simulink library "syntrac_lib"  (R2023b)
settings: Solver=VariableStepAuto  StartTime=0.0  StopTime=10.0  RelTol=1e-3
undefined symbols (not defined in the file or in its folder): aircraft, ic
libraries: unit_conversions_lib x9, actuators_lib x5, vlm_wing_lib x3, flight_parameters_lib x1, axes_transformation_lib x1, rigidBody_lib x1
settings Model: Creator=yannic  LastModifiedBy=Ole Bunde

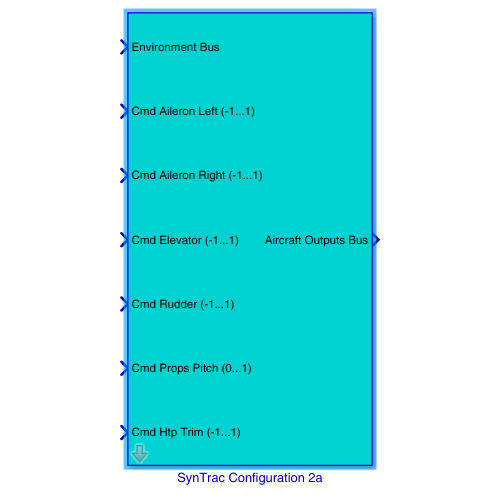
[thumbnail: Simulink's stored preview of the top-level diagram]
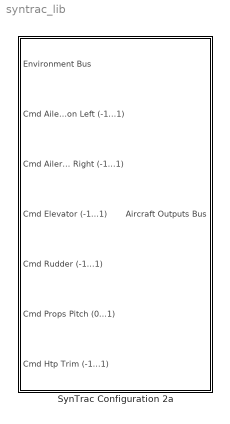
== system syntrac_lib ==
  SynTrac Configuration 2a : Subsystem  mask{aircraft=aircraft, ic=ic}
      mask prompts: aircraft "Aircraft parameters struct, see aircraftSe2aCreate"; ic "Initial conditions struct"
      mask init:
      | aircraft_state = aircraftSyntracGetState(aircraft);
      | struct2bus(aircraft_state);
      mask DialogControl DescGroupVar Prompt: Rigid aircraft with steady aerodynamics
      mask DialogControl DescTextVar Prompt: Rigid-body equations of motion, steady aerodynamics based on nonlinear lifting-line method.

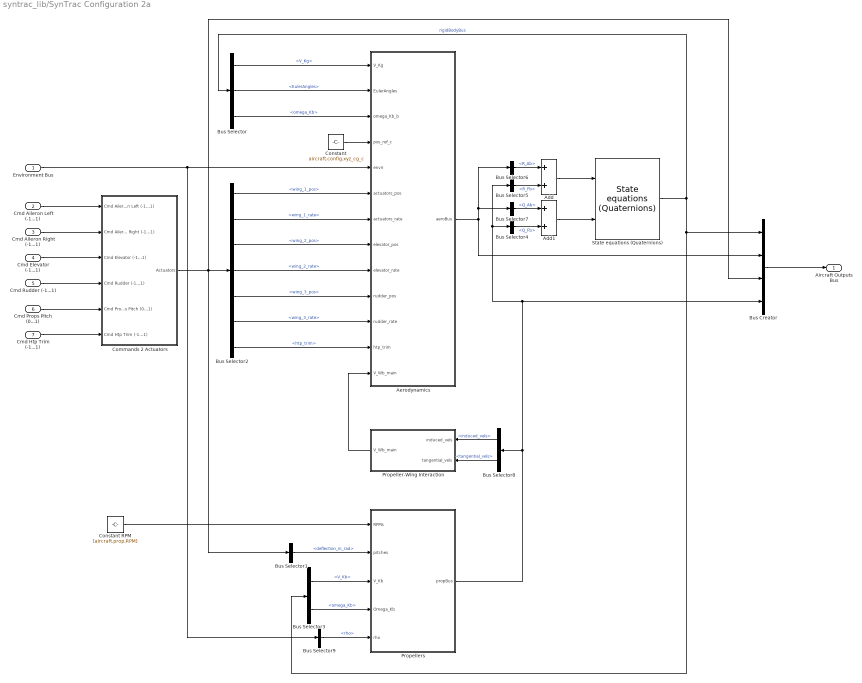
== system syntrac_lib/SynTrac Configuration 2a ==
  Environment Bus : Inport
  Cmd Aileron Left (-1...1) : Inport  Port=2
  Cmd Aileron Right (-1...1) : Inport  Port=3
  Cmd Elevator (-1...1) : Inport  Port=4
  Cmd Rudder (-1...1) : Inport  Port=5
  Cmd Props Pitch (0...1) : Inport  Port=6
  Cmd Htp Trim (-1...1) : Inport  Port=7
  Add : Sum
  Add1 : Sum
  Aerodynamics : Subsystem
  Bus Creator : BusCreator  Inputs=4
  Bus Selector : BusSelector  OutputSignals=V_Kg,EulerAngles,omega_Kb
  Bus Selector1 : BusSelector  OutputSignals=props_pitch.deflection_in_rad
  Bus Selector2 : BusSelector  OutputSignals=wing_1_pos,wing_1_rate,wing_2_pos,wing_2_rate,wing_3_pos,wing_3_rate,htp_trim
  Bus Selector3 : BusSelector  OutputSignals=V_Kb,omega_Kb
  Bus Selector4 : BusSelector  OutputSignals=Q_Fb
  Bus Selector5 : BusSelector  OutputSignals=R_Fb
  Bus Selector6 : BusSelector  OutputSignals=R_Ab
  Bus Selector7 : BusSelector  OutputSignals=Q_Ab
  Bus Selector8 : BusSelector  OutputSignals=induced_vels,tangential_vels
  Bus Selector9 : BusSelector  OutputSignals=atmosphere.rho
  Commands 2 Actuators : Subsystem  mask{aileron=aircraft.actuators.aileron, elevator=aircraft.actuators.elevator, rudder=aircraft.actuators.rudder, prop=aircraft.actuators.prop_pitch, htp_trim=aircraft.actuators.htp_trim, ic=ic.act}
      mask prompts: aileron "Aileron parameters"; elevator "Elevator parameters"; rudder "Rudder parameters"; prop "Engines parameters"; htp_trim "Trimmable horizontal tailplane (htp) parameters"; ic "Initial conditions struct"
      mask DialogControl DescGroupVar Prompt: SE2A Actuator Dynamics
      mask DialogControl DescTextVar Prompt: Input commands are defined as bus.
  Constant : Constant  Value=aircraft.config.xyz_cg_c
  Constant RPM : Constant  Value=[aircraft.prop.RPM]
  Propeller-Wing Interaction : Subsystem  mask{prop=aircraft.prop, wing=aircraft.wing_main}
      mask prompts: prop "Propeller struct"; wing "Wing struct"
  Propellers : Subsystem  mask{prop=aircraft.prop, prop_map=aircraft.prop_table, pos_cg_c=aircraft.config.xyz_cg_c}
      mask prompts: prop "Array of propeller structs"; prop_map "Propeller map struct"; pos_cg_c "Center of gravity positions in c frame, m"
      mask init:
      | num_props = length(prop);
      |     M_bp = zeros(3,3,num_props);
      |     r_p_b = zeros(3,num_props);
      |     for i = 1:num_props
      |         M_bp(:,:,i) = [ ...
      |             cos(prop(i).angle),0,sin(prop(i).angle); ...
      |             0,1,0; ...
      |             -sin(prop(i).angle),0,cos(prop(i).angle) ...
      |             ];
      |         r_p_b(:,i) = prop(i).pos_c - pos_cg_c;
      |     end
      |     prop_ang = [prop.angle];
  State equations (Quaternions) : rigidBody_lib/State equations (Quaternions)  m=aircraft.body.m  I=aircraft.body.I  is_g_checked=off  g=9.81  omega_Kb_0=ic.omega_Kb  q_bg_0=ic.q_bg  V_Kb_0=ic.V_Kb  s_g_0=ic.s_Kg
      settings: SourceProductName=LADAC
  Aircraft Outputs Bus : Outport  VectorParamsAs1DForOutWhenUnconnected=off
  wires:
  Add/1 -> State equations (Quaternions)/1
  Environment Bus/1 -> Aerodynamics/5(envir), Bus Selector9/1
  State equations (Quaternions)/1 -> Bus Creator/1, Bus Selector3/1, Bus Selector/1  "rigidBodyBus"
  Bus Selector/1 -> Aerodynamics/1(V_Kg)  "<V_Kg>"
  Bus Selector/2 -> Aerodynamics/2(EulerAngles)  "<EulerAngles>"
  Bus Selector/3 -> Aerodynamics/3(omega_Kb_b)  "<omega_Kb>"
  Bus Creator/1 -> Aircraft Outputs Bus/1
  Bus Selector2/6 -> Aerodynamics/11(rudder_rate)  "<wing_3_rate>"
  Bus Selector2/7 -> Aerodynamics/12(htp_trim)  "<htp_trim>"
  Bus Selector2/3 -> Aerodynamics/8(elevator_pos)  "<wing_2_pos>"
  Bus Selector2/2 -> Aerodynamics/7(actuators_rate)  "<wing_1_rate>"
  Cmd Aileron Left (-1...1)/1 -> Commands 2 Actuators/1(Cmd Aileron Left (-1...1))
  Bus Selector2/1 -> Aerodynamics/6(actuators_pos)  "<wing_1_pos>"
  Bus Selector2/5 -> Aerodynamics/10(rudder_pos)  "<wing_3_pos>"
  Bus Selector2/4 -> Aerodynamics/9(elevator_rate)  "<wing_2_rate>"
  Constant/1 -> Aerodynamics/4(pos_ref_c)
  Commands 2 Actuators/1(Actuators) -> Bus Selector1/1, Bus Creator/3, Bus Selector2/1
  Cmd Aileron Right (-1...1)/1 -> Commands 2 Actuators/2(Cmd Aileron Right (-1...1))
  Cmd Elevator (-1...1)/1 -> Commands 2 Actuators/3(Cmd Elevator (-1...1))
  Cmd Rudder (-1...1)/1 -> Commands 2 Actuators/4(Cmd Rudder (-1...1))
  Cmd Props Pitch (0...1)/1 -> Commands 2 Actuators/5(Cmd Props Pitch (0...1))
  Cmd Htp Trim (-1...1)/1 -> Commands 2 Actuators/6(Cmd Htp Trim (-1...1))
  Constant RPM/1 -> Propellers/1(RPMs)
  Bus Selector1/1 -> Propellers/2(pitches)  "<deflection_in_rad>"
  Bus Selector3/1 -> Propellers/3(V_Kb)  "<V_Kb>"
  Bus Selector3/2 -> Propellers/4(Omega_Kb)  "<omega_Kb>"
  Add1/1 -> State equations (Quaternions)/2
  Propellers/1(propBus) -> Bus Selector5/1, Bus Selector4/1, Bus Creator/4, Bus Selector8/1
  Bus Selector5/1 -> Add/2  "<R_Fb>"
  Bus Selector4/1 -> Add1/2  "<Q_Fb>"
  Bus Selector6/1 -> Add/1  "<R_Ab>"
  Bus Selector7/1 -> Add1/1  "<Q_Ab>"
  Aerodynamics/1(aeroBus) -> Bus Creator/2, Bus Selector7/1, Bus Selector6/1
  Bus Selector8/1 -> Propeller-Wing Interaction/1(induced_vels)  "<induced_vels>"
  Bus Selector9/1 -> Propellers/5(rho)  "<rho>"
  Bus Selector8/2 -> Propeller-Wing Interaction/2(tangential_vels)  "<tangential_vels>"
  Propeller-Wing Interaction/1(V_Wb_main) -> Aerodynamics/13(V_Wb_main)

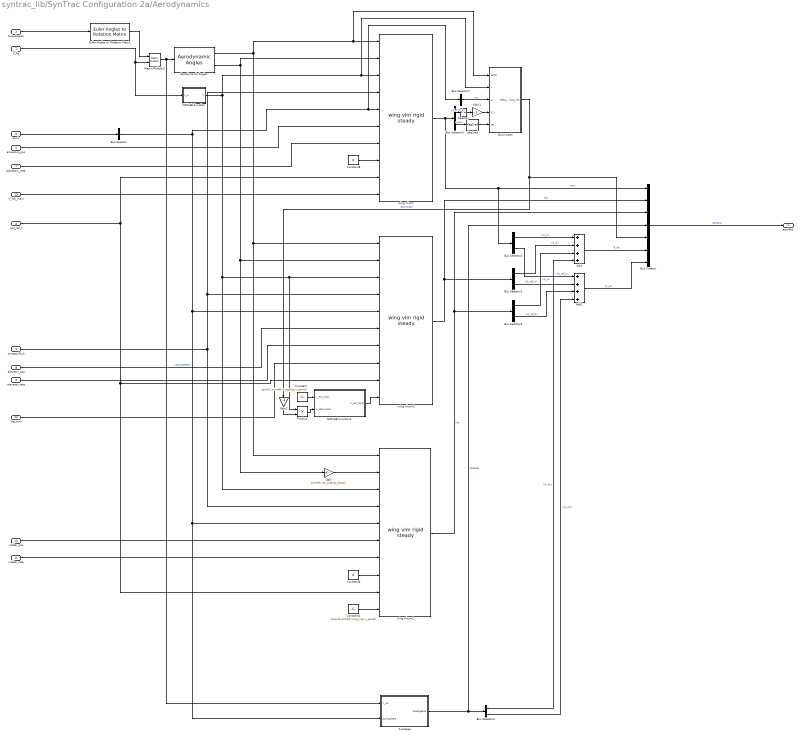
== system syntrac_lib/SynTrac Configuration 2a/Aerodynamics ==
  V_Kg : Inport
  EulerAngles : Inport  Port=2
  omega_Kb_b : Inport  Port=3
  pos_ref_c : Inport  Port=4
  envir : Inport  Port=5
  actuators_pos : Inport  Port=6
  actuators_rate : Inport  Port=7
  elevator_pos : Inport  Port=8
  elevator_rate : Inport  Port=9
  rudder_pos : Inport  Port=10
  rudder_rate : Inport  Port=11
  htp_trim : Inport  Port=12
  V_Wb_main : Inport  Port=13
  Add : Sum  Inputs=++++
  Add1 : Sum  Inputs=++++
  Aerodynamic Angles : flight_parameters_lib/Aerodynamic Angles  SystemSampleTime=-1  VariantActivationTime=update diagram  AllowFlexibleInterface=on  Latency=0  AutoFrameSizeCalculation=off
      settings: SourceProductName=LADAC
  Bus Creator : BusCreator  Inputs=7
  Bus Selector : BusSelector  OutputSignals=atmosphere
  Bus Selector1 : BusSelector  OutputSignals=aero.force_glob.R_b,aero.force_glob.Q_ref_b
  Bus Selector2 : BusSelector  OutputSignals=aero.force_glob.R_b,aero.force_glob.Q_ref_b
  Bus Selector3 : BusSelector  OutputSignals=aero.force_glob.R_b,aero.force_glob.Q_ref_b
  Bus Selector4 : BusSelector  OutputSignals=R_Ab,Q_Ab
  Bus Selector5 : BusSelector  OutputSignals=aero.coeff_glob.C_XYZ_b,actuators.pos
  Bus Selector7 : BusSelector  OutputSignals=a
  Constant : Constant  Value=zeros(3,aircraft.wing_htp.n_panel)
  Constant2 : Constant  Value=zeros(3,aircraft.wing_vtp.n_panel)
  Constant6 : Constant  Value=0
  Constant8 : Constant  Value=0
  Downwash : Subsystem
  Euler Angles to Rotation Matrix : axes_transformation_lib/Euler Angles to Rotation Matrix  SystemSampleTime=-1  VariantActivationTime=update diagram  AllowFlexibleInterface=on  Latency=0  AutoFrameSizeCalculation=off
      settings: SourceProductName=LADAC
  Fuselage : Subsystem
  Gain : Gain  Gain=aircraft.vtp_sideslip_factor
  Gain1 : Gain  Gain=-1
  Gain2 : Gain  Gain=-1
  MATLAB Function : MATLAB Function  TreatAsAtomicUnit=on
  MATLAB Function4 : MATLAB Function  TreatAsAtomicUnit=on
  MatrixMultiply2 : Product  Multiplication=Matrix(*)
  Product : Product
  Selector : Selector  InputPortWidth=3  IndexOptions=Index vector (dialog)  Indices=3  OutputSizes=1
  deg2rad : unit_conversions_lib/deg2rad
      settings: SourceProductName=LADAC
  wing nlvsm : vlm_wing_lib/wing vlm rigid steady  wing_struct=aircraft.wing_main  wing_state_bus=wing_1_state_bus  alpha_ind_init=0
      settings: SourceProductName=LADAC
  wing nlvsm1 : vlm_wing_lib/wing vlm rigid steady  wing_struct=aircraft.wing_htp  wing_state_bus=wing_2_state_bus  alpha_ind_init=0
      settings: SourceProductName=LADAC
  wing nlvsm2 : vlm_wing_lib/wing vlm rigid steady  wing_struct=aircraft.wing_vtp  wing_state_bus=wing_3_state_bus  alpha_ind_init=0
      settings: SourceProductName=LADAC
  aeroBus : Outport  VectorParamsAs1DForOutWhenUnconnected=off
  wires:
  Euler Angles to Rotation Matrix/1 -> MatrixMultiply2/1
  EulerAngles/1 -> Euler Angles to Rotation Matrix/1
  Aerodynamic Angles/1 -> wing nlvsm2/1, wing nlvsm1/1, Downwash/1(alpha), wing nlvsm/1
  Bus Selector/1 -> wing nlvsm/5, Bus Selector7/1, Fuselage/2(atmosphere), wing nlvsm2/5, wing nlvsm1/5  "<atmosphere>"
  Add/1 -> Bus Creator/6  "R_Ab"
  Add1/1 -> Bus Creator/7  "Q_Ab"
  V_Kg/1 -> MATLAB Function/1(V_A), MatrixMultiply2/2
  MatrixMultiply2/1 -> Fuselage/1(V_Ab), Aerodynamic Angles/1
  Bus Selector1/2 -> Add1/2  "<Q_ref_b>"
  Bus Selector1/1 -> Add/2  "<R_b>"
  elevator_pos/1 -> wing nlvsm1/6
  htp_trim/1 -> wing nlvsm1/8
  Bus Creator/1 -> aeroBus/1  "aeroBus"
  actuators_pos/1 -> wing nlvsm/6
  Constant6/1 -> wing nlvsm/8
  Bus Selector2/1 -> Add/1  "<R_b>"
  Bus Selector2/2 -> Add1/1  "<Q_ref_b>"
  rudder_pos/1 -> wing nlvsm2/6
  Constant8/1 -> wing nlvsm2/8
  pos_ref_c/1 -> wing nlvsm/9, wing nlvsm2/9, wing nlvsm1/9
  wing nlvsm2/1 -> Bus Creator/3, Bus Selector3/1  "vtp"
  Bus Selector3/1 -> Add/3  "<R_b>"
  Bus Selector3/2 -> Add1/3  "<Q_ref_b>"
  omega_Kb_b/1 -> wing nlvsm/4, wing nlvsm1/4, wing nlvsm2/4
  wing nlvsm1/1 -> Bus Creator/2, Bus Selector1/1  "htp"
  rudder_rate/1 -> wing nlvsm2/7
  actuators_rate/1 -> wing nlvsm/7
  elevator_rate/1 -> wing nlvsm1/7
  Fuselage/1(fuselageBus) -> Bus Creator/4, Bus Selector4/1  "fuselage"
  Bus Selector4/1 -> Add/4  "<R_Ab>"
  Bus Selector4/2 -> Add1/4  "<Q_Ab>"
  Aerodynamic Angles/2 -> Gain/1, wing nlvsm1/2, wing nlvsm/2
  Gain/1 -> wing nlvsm2/2
  MATLAB Function/1(V) -> wing nlvsm/3, Downwash/2(V), wing nlvsm2/3, wing nlvsm1/3, Product/1
  MATLAB Function4/1(V_ext_local) -> wing nlvsm1/10
  wing nlvsm/1 -> Bus Selector5/1, Bus Selector2/1, Bus Creator/1  "main"
  envir/1 -> Bus Selector/1
  Constant/1 -> MATLAB Function4/1("V_ext_local ")
  Constant2/1 -> wing nlvsm2/10
  V_Wb_main/1 -> wing nlvsm/10
  Bus Selector7/1 -> Downwash/3(a)  "<a>"
  Bus Selector5/1 -> Selector/1  "<C_XYZ_b>"
  Bus Selector5/2 -> deg2rad/1  "<pos>"
  Downwash/1(Delta_alpha_htp) -> Gain2/1, Bus Creator/5  "downwash"
  Product/1 -> MATLAB Function4/2(w_downwash)
  Selector/1 -> Gain1/1
  Gain1/1 -> Downwash/4(C_L)
  Gain2/1 -> Product/2
  deg2rad/1 -> Downwash/5(eta)

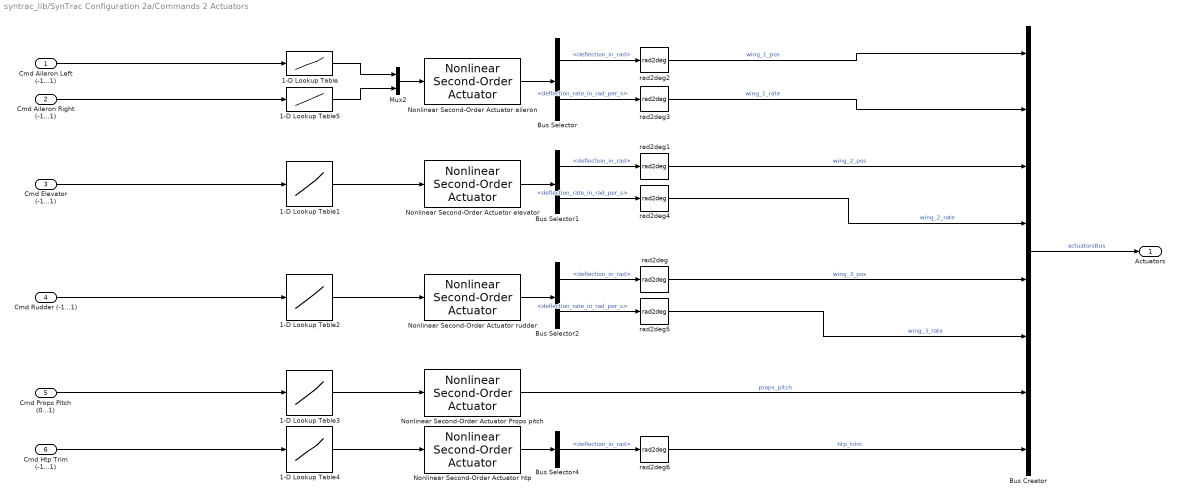
== system syntrac_lib/SynTrac Configuration 2a/Commands 2 Actuators ==
  Cmd Aileron Left (-1...1) : Inport
  Cmd Aileron Right (-1...1) : Inport  Port=2
  Cmd Elevator (-1...1) : Inport  Port=3
  Cmd Rudder (-1...1) : Inport  Port=4
  Cmd Props Pitch (0...1) : Inport  Port=5
  Cmd Htp Trim (-1...1) : Inport  Port=6
  1-D Lookup Table : Lookup_n-D  NumberOfTableDimensions=1  BreakpointsForDimension1=[-1,1]  Table=[aileron.defl_min,aileron.defl_max]  ExtrapMethod=Clip  InternalRulePriority=Speed  RndMeth=Simplest
  1-D Lookup Table1 : Lookup_n-D  NumberOfTableDimensions=1  BreakpointsForDimension1=[-1,1]  Table=[elevator.defl_min,elevator.defl_max]  ExtrapMethod=Clip  InternalRulePriority=Speed  RndMeth=Simplest
  1-D Lookup Table2 : Lookup_n-D  NumberOfTableDimensions=1  BreakpointsForDimension1=[-1,1]  Table=[rudder.defl_min,rudder.defl_max]  ExtrapMethod=Clip  InternalRulePriority=Speed  RndMeth=Simplest
  1-D Lookup Table3 : Lookup_n-D  NumberOfTableDimensions=1  BreakpointsForDimension1=[0,1]  Table=[prop.defl_min,prop.defl_max]  ExtrapMethod=Clip  InternalRulePriority=Speed  RndMeth=Simplest
  1-D Lookup Table4 : Lookup_n-D  NumberOfTableDimensions=1  BreakpointsForDimension1=[-1,1]  Table=[htp_trim.defl_min,htp_trim.defl_max]  ExtrapMethod=Clip  InternalRulePriority=Speed  RndMeth=Simplest
  1-D Lookup Table5 : Lookup_n-D  NumberOfTableDimensions=1  BreakpointsForDimension1=[-1,1]  Table=[aileron.defl_min,aileron.defl_max]  ExtrapMethod=Clip  InternalRulePriority=Speed  RndMeth=Simplest
  Bus Creator : BusCreator  Inputs=8
  Bus Selector : BusSelector  OutputSignals=deflection_in_rad,deflection_rate_in_rad_per_s
  Bus Selector1 : BusSelector  OutputSignals=deflection_in_rad,deflection_rate_in_rad_per_s
  Bus Selector2 : BusSelector  OutputSignals=deflection_in_rad,deflection_rate_in_rad_per_s
  Bus Selector4 : BusSelector  OutputSignals=deflection_in_rad
  Mux2 : Mux  Inputs=2
  Nonlinear Second-Order Actuator Props pitch : actuators_lib/Nonlinear Second-Order Actuator  omega=prop.omega  d=prop.D  A_max=prop.defl_max  A_min=prop.defl_min  dot_A_max=prop.defl_rate_max  dot_A_min=prop.defl_rate_min  A_0=ic.prop  dot_A_0=0
      settings: SourceProductName=LADAC
  Nonlinear Second-Order Actuator aileron : actuators_lib/Nonlinear Second-Order Actuator  omega=aileron.omega  d=aileron.D  A_max=aileron.defl_max  A_min=aileron.defl_min  dot_A_max=aileron.defl_rate_max  dot_A_min=aileron.defl_rate_min  A_0=ic.aileron  dot_A_0=0
      settings: SourceProductName=LADAC
  Nonlinear Second-Order Actuator elevator : actuators_lib/Nonlinear Second-Order Actuator  omega=elevator.omega  d=elevator.D  A_max=elevator.defl_max  A_min=elevator.defl_min  dot_A_max=elevator.defl_rate_max  dot_A_min=elevator.defl_rate_min  A_0=ic.elevator  dot_A_0=0
      settings: SourceProductName=LADAC
  Nonlinear Second-Order Actuator htp : actuators_lib/Nonlinear Second-Order Actuator  omega=htp_trim.omega  d=htp_trim.D  A_max=htp_trim.defl_max  A_min=htp_trim.defl_min  dot_A_max=htp_trim.defl_rate_max  dot_A_min=htp_trim.defl_rate_min  A_0=ic.htp_trim  dot_A_0=0
      settings: SourceProductName=LADAC
  Nonlinear Second-Order Actuator rudder : actuators_lib/Nonlinear Second-Order Actuator  omega=rudder.omega  d=rudder.D  A_max=rudder.defl_max  A_min=rudder.defl_min  dot_A_max=rudder.defl_rate_max  dot_A_min=rudder.defl_rate_min  A_0=ic.rudder  dot_A_0=0
      settings: SourceProductName=LADAC
  rad2deg{,1..6} (7 alike) : unit_conversions_lib/rad2deg
      settings: SourceProductName=LADAC
  Actuators : Outport  VectorParamsAs1DForOutWhenUnconnected=off
  wires:
  Mux2/1 -> Nonlinear Second-Order Actuator aileron/1
  1-D Lookup Table5/1 -> Mux2/2
  1-D Lookup Table4/1 -> Nonlinear Second-Order Actuator htp/1
  rad2deg6/1 -> Bus Creator/8  "htp_trim"
  Nonlinear Second-Order Actuator htp/1 -> Bus Selector4/1
  Bus Selector4/1 -> rad2deg6/1  "<deflection_in_rad>"
  Cmd Htp Trim (-1...1)/1 -> 1-D Lookup Table4/1
  Nonlinear Second-Order Actuator Props pitch/1 -> Bus Creator/7  "props_pitch"
  1-D Lookup Table3/1 -> Nonlinear Second-Order Actuator Props pitch/1
  Cmd Props Pitch (0...1)/1 -> 1-D Lookup Table3/1
  Cmd Aileron Right (-1...1)/1 -> 1-D Lookup Table5/1
  Cmd Aileron Left (-1...1)/1 -> 1-D Lookup Table/1
  rad2deg5/1 -> Bus Creator/6  "wing_3_rate"
  Bus Selector2/2 -> rad2deg5/1  "<deflection_rate_in_rad_per_s>"
  rad2deg4/1 -> Bus Creator/4  "wing_2_rate"
  rad2deg3/1 -> Bus Creator/2  "wing_1_rate"
  Bus Selector1/2 -> rad2deg4/1  "<deflection_rate_in_rad_per_s>"
  Bus Selector/2 -> rad2deg3/1  "<deflection_rate_in_rad_per_s>"
  1-D Lookup Table2/1 -> Nonlinear Second-Order Actuator rudder/1
  Cmd Rudder (-1...1)/1 -> 1-D Lookup Table2/1
  1-D Lookup Table1/1 -> Nonlinear Second-Order Actuator elevator/1
  Cmd Elevator (-1...1)/1 -> 1-D Lookup Table1/1
  1-D Lookup Table/1 -> Mux2/1
  Bus Selector2/1 -> rad2deg/1  "<deflection_in_rad>"
  Bus Selector1/1 -> rad2deg1/1  "<deflection_in_rad>"
  Nonlinear Second-Order Actuator aileron/1 -> Bus Selector/1
  Nonlinear Second-Order Actuator rudder/1 -> Bus Selector2/1
  Nonlinear Second-Order Actuator elevator/1 -> Bus Selector1/1
  Bus Selector/1 -> rad2deg2/1  "<deflection_in_rad>"
  rad2deg/1 -> Bus Creator/5  "wing_3_pos"
  rad2deg1/1 -> Bus Creator/3  "wing_2_pos"
  rad2deg2/1 -> Bus Creator/1  "wing_1_pos"
  Bus Creator/1 -> Actuators/1  "actuatorsBus"

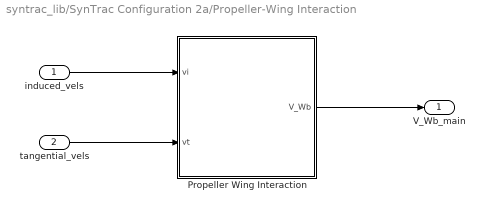
== system syntrac_lib/SynTrac Configuration 2a/Propeller-Wing Interaction ==
  induced_vels : Inport
  tangential_vels : Inport  Port=2
  Propeller Wing Interaction : MATLAB Function  TreatAsAtomicUnit=on
  V_Wb_main : Outport
  wires:
  Propeller Wing Interaction/1(V_Wb) -> V_Wb_main/1
  induced_vels/1 -> Propeller Wing Interaction/1(vi)
  tangential_vels/1 -> Propeller Wing Interaction/2(vt)

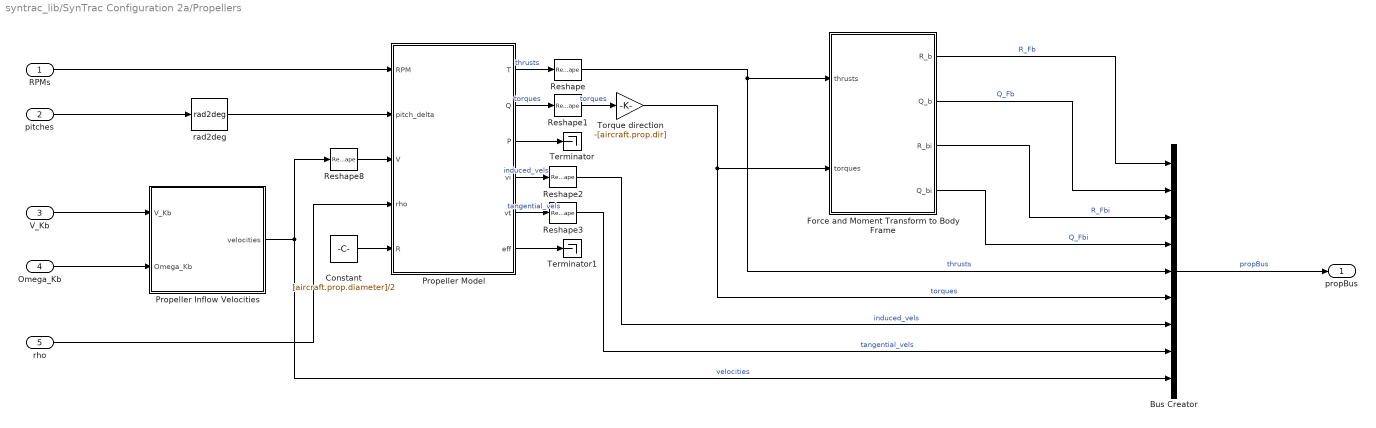
== system syntrac_lib/SynTrac Configuration 2a/Propellers ==
  RPMs : Inport
  pitches : Inport  Port=2
  V_Kb : Inport  Port=3
  Omega_Kb : Inport  Port=4
  rho : Inport  Port=5
  Bus Creator : BusCreator  Inputs=9
  Constant : Constant  Value=[aircraft.prop.diameter]/2
  Force and Moment Transform to Body Frame : MATLAB Function  TreatAsAtomicUnit=on
  Propeller Inflow Velocities : MATLAB Function  TreatAsAtomicUnit=on
  Propeller Model : MATLAB Function  TreatAsAtomicUnit=on
  Reshape{,1..3} (4 alike) : Reshape  OutputDimensionality=Row vector (2-D)
  Reshape8 : Reshape
  Terminator : Terminator
  Terminator1 : Terminator
  Torque direction : Gain  Gain=-[aircraft.prop.dir]
  rad2deg : unit_conversions_lib/rad2deg
      settings: SourceProductName=LADAC
  propBus : Outport
  wires:
  Reshape8/1 -> Propeller Model/3(V)
  pitches/1 -> rad2deg/1
  Reshape2/1 -> Bus Creator/7  "induced_vels"
  V_Kb/1 -> Propeller Inflow Velocities/1(V_Kb)
  Torque direction/1 -> Bus Creator/6, Force and Moment Transform to Body Frame/2(torques)  "torques"
  Reshape/1 -> Bus Creator/5, Force and Moment Transform to Body Frame/1(thrusts)  "thrusts"
  RPMs/1 -> Propeller Model/1(RPM)
  Omega_Kb/1 -> Propeller Inflow Velocities/2(Omega_Kb)
  Reshape1/1 -> Torque direction/1  "torques"
  Force and Moment Transform to Body Frame/2(Q_b) -> Bus Creator/2  "Q_Fb"
  Force and Moment Transform to Body Frame/1(R_b) -> Bus Creator/1  "R_Fb"
  Propeller Inflow Velocities/1(velocities) -> Reshape8/1, Bus Creator/9  "velocities"
  Bus Creator/1 -> propBus/1  "propBus"
  Force and Moment Transform to Body Frame/3(R_bi) -> Bus Creator/3  "R_Fbi"
  Force and Moment Transform to Body Frame/4(Q_bi) -> Bus Creator/4  "Q_Fbi"
  Reshape3/1 -> Bus Creator/8  "tangential_vels"
  rho/1 -> Propeller Model/4(rho)
  Propeller Model/3(P) -> Terminator/1
  Propeller Model/6(eff) -> Terminator1/1
  Constant/1 -> Propeller Model/5(R)
  Propeller Model/1(T) -> Reshape/1  "thrusts"
  Propeller Model/2(Q) -> Reshape1/1  "torques"
  Propeller Model/4(vi) -> Reshape2/1  "induced_vels"
  Propeller Model/5(vt) -> Reshape3/1  "tangential_vels"
  rad2deg/1 -> Propeller Model/2(pitch_delta)

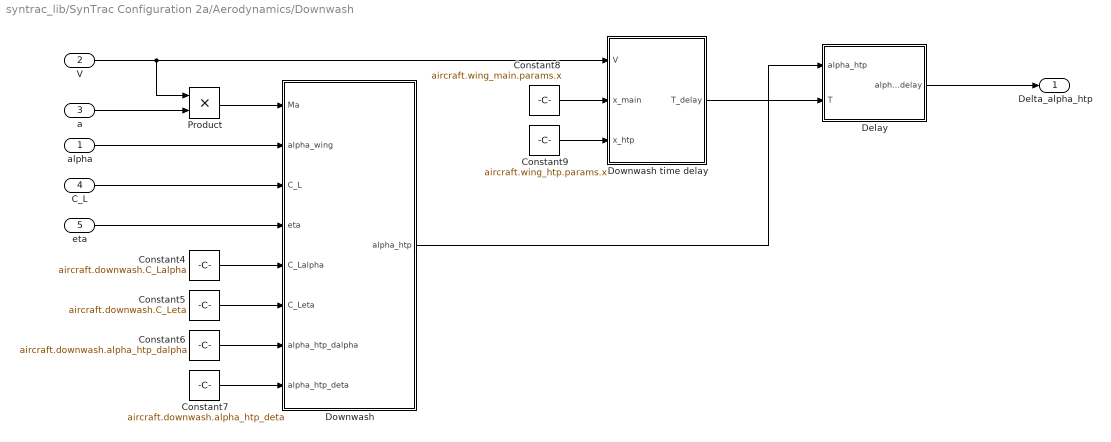
== system syntrac_lib/SynTrac Configuration 2a/Aerodynamics/Downwash ==
  alpha : Inport
  V : Inport  Port=2
  a : Inport  Port=3
  C_L : Inport  Port=4
  eta : Inport  Port=5
  Constant4 : Constant  Value=aircraft.downwash.C_Lalpha
  Constant5 : Constant  Value=aircraft.downwash.C_Leta
  Constant6 : Constant  Value=aircraft.downwash.alpha_htp_dalpha
  Constant7 : Constant  Value=aircraft.downwash.alpha_htp_deta
  Constant8 : Constant  Value=aircraft.wing_main.params.x
  Constant9 : Constant  Value=aircraft.wing_htp.params.x
  Delay : Subsystem
  Downwash : MATLAB Function  TreatAsAtomicUnit=on
  Downwash time delay : MATLAB Function  TreatAsAtomicUnit=on
  Product : Product
  Delta_alpha_htp : Outport  VectorParamsAs1DForOutWhenUnconnected=off
  wires:
  Constant7/1 -> Downwash/8(alpha_htp_deta)
  Constant5/1 -> Downwash/6(C_Leta)
  Constant6/1 -> Downwash/7(alpha_htp_dalpha)
  Constant4/1 -> Downwash/5(C_Lalpha)
  C_L/1 -> Downwash/3(C_L)
  Constant8/1 -> Downwash time delay/2(x_main)
  Constant9/1 -> Downwash time delay/3(x_htp)
  eta/1 -> Downwash/4(eta)
  V/1 -> Downwash time delay/1(V), Product/1
  Downwash time delay/1(T_delay) -> Delay/2(T)
  Downwash/1(alpha_htp) -> Delay/1(alpha_htp)
  Delay/1(alpha_htp_delay) -> Delta_alpha_htp/1
  a/1 -> Product/2
  alpha/1 -> Downwash/2(alpha_wing)
  Product/1 -> Downwash/1(Ma)

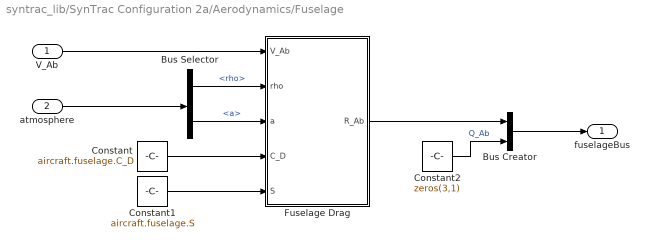
== system syntrac_lib/SynTrac Configuration 2a/Aerodynamics/Fuselage ==
  V_Ab : Inport
  atmosphere : Inport  Port=2
  Bus Creator : BusCreator  Inputs=2
  Bus Selector : BusSelector  OutputSignals=rho,a
  Constant : Constant  Value=aircraft.fuselage.C_D
  Constant1 : Constant  Value=aircraft.fuselage.S
  Constant2 : Constant  Value=zeros(3,1)  VectorParams1D=off
  Fuselage Drag : MATLAB Function  TreatAsAtomicUnit=on
  fuselageBus : Outport
  wires:
  V_Ab/1 -> Fuselage Drag/1(V_Ab)
  atmosphere/1 -> Bus Selector/1
  Bus Selector/1 -> Fuselage Drag/2(rho)  "<rho>"
  Bus Selector/2 -> Fuselage Drag/3(a)  "<a>"
  Fuselage Drag/1(R_Ab) -> Bus Creator/1
  Constant/1 -> Fuselage Drag/4(C_D)
  Constant1/1 -> Fuselage Drag/5(S)
  Bus Creator/1 -> fuselageBus/1
  Constant2/1 -> Bus Creator/2  "Q_Ab"

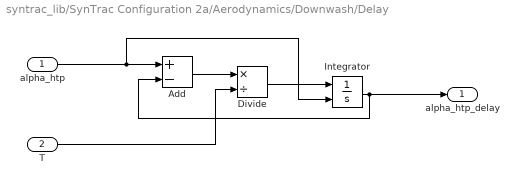
== system syntrac_lib/SynTrac Configuration 2a/Aerodynamics/Downwash/Delay ==
  alpha_htp : Inport
  T : Inport  Port=2
  Add : Sum  Inputs=+-
  Divide : Product  Inputs=*/
  Integrator : Integrator  InitialConditionSource=external
  alpha_htp_delay : Outport
  wires:
  alpha_htp/1 -> Integrator/2, Add/1
  Add/1 -> Divide/1
  Divide/1 -> Integrator/1
  Integrator/1 -> alpha_htp_delay/1, Add/2
  T/1 -> Divide/2

== matlab function syntrac_lib/SynTrac Configuration 2a/Aerodynamics/Downwash/Downwash time delay ==
  data: V input; x_main input; T_delay output; x_htp input
function T_delay = fcn(V, x_main, x_htp)
T_delay = divideFinite( x_main - x_htp, V );
% avoid singularity
T_delay(T_delay<0.001) = 0.001;
end

== matlab function syntrac_lib/SynTrac Configuration 2a/Aerodynamics/Fuselage/Fuselage Drag ==
  data: V_Ab input; R_Ab output; rho input; a input; C_D input; S input
function R_Ab = fcn(V_Ab, rho, a, C_D, S)
%#codegen
V_A = norm(V_Ab);
n_A = V_Ab/V_A;
Ma = V_A/a;
D_0 = C_D * rho/2*V_A^2*S;
D = D_0 * 1/sqrt(1-Ma^2);
R_Ab = zeros(3,1);
R_Ab(:) = -D*n_A;
end

== matlab function syntrac_lib/SynTrac Configuration 2a/Propeller-Wing Interaction/Propeller Wing Interaction ==
  data: V_Wb output; vi input; vt input; prop parameter; wing parameter
function V_Wb = propellerWingInteraction( vi, vt, prop, wing )

% Propeller slipstream
prop_pos = [prop.pos_c];
prop_y_pos = prop_pos(2,:);
V_Wb = wingApplySlipstream( wing, prop_y_pos, [prop.angle], ...
    [prop.diameter], vi, vt, [prop.dir], [prop.k_vi], ...
    [prop.k_vt] );

end

== matlab function syntrac_lib/SynTrac Configuration 2a/Aerodynamics/MATLAB Function ==
  data: V_A input; V output
function V = fcn(V_A)
V = norm(V_A,2);
end

== matlab function syntrac_lib/SynTrac Configuration 2a/Propellers/Force and Moment Transform to Body Frame ==
  data: thrusts input; torques input; R_b output; Q_b output; r_p_b parameter; R_bi output; Q_bi output; prop_ang parameter
function [R_b,Q_b,R_bi,Q_bi] = fcn(thrusts, torques, r_p_b, prop_ang)

num_props = length(thrusts);
R_p = [ thrusts.*cos(prop_ang); zeros(1,num_props); thrusts.*sin(-prop_ang) ];
Q_p = [ torques(:)'.*cos(prop_ang); zeros(1,num_props); torques(:)'.*sin(-prop_ang) ];

[ R_bi, Q_bi ] = forceMomentTransform( R_p, Q_p, r_p_b, eye(3) );

R_b = sum(R_bi,2);
Q_b = sum(Q_bi,2);

end

== matlab function syntrac_lib/SynTrac Configuration 2a/Propellers/Propeller Inflow Velocities ==
  data: V_Kb input; velocities output; Omega_Kb input; r_p_b parameter; M_bp parameter
function velocities = fcn(V_Kb, Omega_Kb, r_p_b, M_bp)
num_props = size(r_p_b,2);
velocities = zeros(1,num_props);
for i = 1:num_props
    V_p = velocityAndRateTransform(V_Kb, Omega_Kb, r_p_b(:,i), M_bp(:,:,i)');
    velocities(i) = V_p(1);
end

== matlab function syntrac_lib/SynTrac Configuration 2a/Propellers/Propeller Model ==
  data: T output; RPM input; pitch_delta input; V input; rho input; R input; Q output; P output; vi output; vt output; eff output; prop_map parameter
function [T, Q, P, vi, vt, eff] = ...
    propeller_model(RPM, pitch_delta, V, rho, R, prop_map)

[T, Q, P, vi, ~, vt, eff] = ...
    propeller_model_sfcn(prop_map, RPM, pitch_delta, V, rho, R);

end

== matlab function syntrac_lib/SynTrac Configuration 2a/Aerodynamics/MATLAB Function4 ==
  data: V_ext_local input; V_ext_local output; w_downwash input
function V_ext_local  = fcn(V_ext_local ,w_downwash)

V_ext_local(3,:) = V_ext_local(3,:) + w_downwash;

end

== matlab function syntrac_lib/SynTrac Configuration 2a/Aerodynamics/Downwash/Downwash ==
  data: Ma input; alpha_wing input; alpha_htp output; C_L input; eta input; C_Lalpha input; C_Leta input; alpha_htp_dalpha input; alpha_htp_deta input
function alpha_htp  = fcn(Ma, alpha_wing, C_L, eta, C_Lalpha, C_Leta, alpha_htp_dalpha, alpha_htp_deta)
comp = divideFinite(1,sqrtReal(abs(1-Ma*Ma)));
C_L_eta = comp*C_Leta(:) .* eta(:);
C_L_alpha = mean(C_L) - sum(C_L_eta);
% downwash due to main wing lift
alpha = C_L_alpha / C_Lalpha;
alpha_htp = alpha_htp_dalpha(:)' * alpha;
% add downwash due to main wing flap deflections
alpha_htp = alpha_htp + sum(alpha_htp_deta(:)' .* eta);
% reduce downwash in case of high aerodynamic angles
cos_arg = 3 * pi/2*(1-cos(alpha_wing));
cos_arg(abs(cos_arg)>pi/2) = pi/2;    
alpha_htp = alpha_htp * cos(cos_arg);
end
